simulink model "baseline_A_inference_v5"  (R2026a)
settings: Solver=FixedStepDiscrete  StartTime=0  StopTime=23  FixedStep=1
model workspace (MAT data in the model file):
  baseline_arch = 1
  baseline_inputs = timeseries
  baseline_inputs.Name = 'unnamed'
  baseline_inputs.DataInfo = tsdata.datametadata
  baseline_inputs.DataInfo.Interpolation = tsdata.interpolation
  baseline_inputs.DataInfo.Interpolation.Fhandle : function handle (value not decoded)
  baseline_inputs.DataInfo.Interpolation.Name = 'linear'
  baseline_inputs.TimeInfo = tsdata.timemetadata
  baseline_inputs.TimeInfo.Length = 24
  baseline_inputs.TimeInfo.DuplicateTimes = 0
  baseline_inputs.TimeInfo.Time_ = [0; 1; 2; 3; 4; 5; 6; 7; 8; 9; 10; 11; 12; 13; 14; 15; 16; 17; 18; 19; 20; 21; 22; 23]
  baseline_inputs.TimeInfo.Initialized = 1
  baseline_inputs.QualityInfo = tsdata.qualmetadata
  baseline_inputs.Data_ = [3026.659  81.2  1  2; 2218.177  78.3  1  2; 2902.304  81  1  2; 2193.91933333  77.9  1  2; 2808.14466667  81.3  1  2; 2120.17766667  75.1  1  2; 3824.575  80  1  2; 2700.98066667  75.7  1  2; 3026.659  81.2  1  3; 2205.66033333  74.9  1  3; 2902.304  81  1  3; 2112.29733333  72.9  1  3; 2808.14466667  81.3  1  3; 2092.628  71.7  1  3; 3824.575  80  1  3; 2542.90933333  73.8  1  3; 3026.659  81.2  1  4; 3382.50466667  75  1  4; 2902.304  81  1  4; 2413.05233333  73.3  1  4; 2808.14466667  81.3  1  4; 2538.15333333  73  1  4; 3824.575  80  1  4; 3938.38166667  73.7  1  4]
  baseline_mu = [2625.56568519 77.2222222222]
  baseline_p = [0.666654751449; 0.226875085596; -1.47953239563; 0.274529911025; -0.813940147404; -0.384768139912; 1.63750357072; -1.04590625677; 0.818587516624; -0.172278212697; -0.255378936098; -0.34034588768; 0; 0; 0; 0; 0; 0; 0; 0; 0; 0; 0; 0; 0; 0; 0; 0; 0; 0; 0; 0]
  baseline_sd = [585.088406321 4.03273116323]
Description:
  | Frozen A inference: linear/no-replay/seed101/stage3 demonstration with24 reporting views. Tick=record order, not physical time. Full30-checkpoint parity is in the separate result. No online learning.
settings Model: Creator=salih  LastModifiedBy=salih

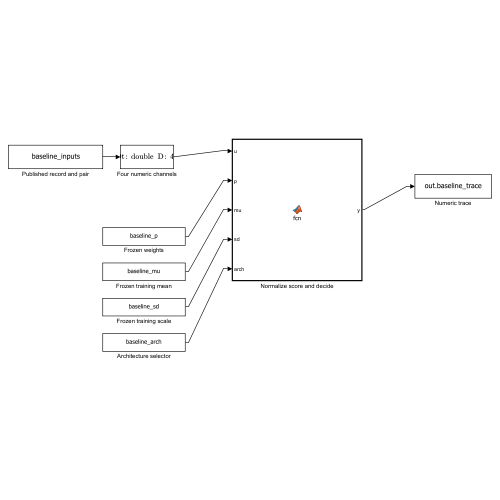
[thumbnail: Simulink's stored preview of the top-level diagram]
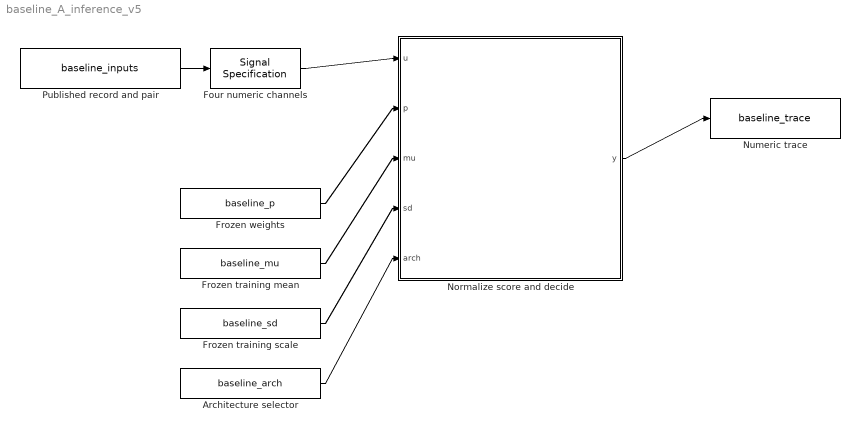
== system baseline_A_inference_v5 ==
  Architecture selector : Constant  Value=baseline_arch
  Four numeric channels : SignalSpecification  OutDataTypeStr=double  Dimensions=4
  Frozen training mean : Constant  Value=baseline_mu
  Frozen training scale : Constant  Value=baseline_sd
  Frozen weights : Constant  Value=baseline_p
  Normalize score and decide : MATLAB Function  TreatAsAtomicUnit=on
  Numeric trace : ToWorkspace  VariableName=baseline_trace  SampleTime=1
  Published record and pair : FromWorkspace  VariableName=baseline_inputs  SampleTime=1  Interpolate=off  OutputAfterFinalValue=Holding final value
  wires:
  Published record and pair/1 -> Four numeric channels/1
  Four numeric channels/1 -> Normalize score and decide/1(u)
  Frozen weights/1 -> Normalize score and decide/2(p)
  Frozen training mean/1 -> Normalize score and decide/3(mu)
  Frozen training scale/1 -> Normalize score and decide/4(sd)
  Architecture selector/1 -> Normalize score and decide/5(arch)
  Normalize score and decide/1(y) -> Numeric trace/1

== matlab function baseline_A_inference_v5/Normalize score and decide ==
  data: u input; y output; p input; mu input; sd input; arch input
function y = fcn(u,p,mu,sd,arch)
%#codegen
% u: [E_MPa, ShoreD, candidate_a, candidate_b]. Pair is control, not a feature.
% p: fixed32 parameter slots. arch1 linear; arch2 two-four-four tanh.
% y: Xnorm2, logits4, probabilities4, margin, forced, selected, status.
% status1 selected,0 nonselection,-1 failure. True label never enters here.
y=nan(1,14); y(12:13)=0; y(14)=-1;
if any(~isfinite(u(:))) || any(~isfinite(p(:))) || ...
        any(~isfinite(mu(:))) || any(~isfinite(sd(:))) || any(sd(:)<=0)
    return;
end
a=u(3); b=u(4);
if a~=1 || b~=floor(b) || b<2 || b>4 || (arch~=1 && arch~=2)
    return;
end
x=[(u(1)-mu(1))/sd(1),(u(2)-mu(2))/sd(2)];
if arch==1
    W=reshape(p(1:8),2,4); bias=reshape(p(9:12),1,4);
    z=x*W+bias;
else
    W1=reshape(p(1:8),2,4); b1=reshape(p(9:12),1,4);
    W2=reshape(p(13:28),4,4); b2=reshape(p(29:32),1,4);
    z=tanh(x*W1+b1)*W2+b2;
end
if any(~isfinite(z)), return; end
m=max(z(a),z(b)); ea=exp(z(a)-m); eb=exp(z(b)-m);
P=zeros(1,4); P(a)=ea/(ea+eb); P(b)=eb/(ea+eb);
margin=abs(P(a)-P(b)); forced=a;
if P(b)>P(a), forced=b; end % accepted pairs ascending; tie -> smallest index
selected=0; status=0;
if margin>=0.15 && P(a)~=P(b), selected=forced; status=1; end
y=[x,z,P,margin,forced,selected,status];
end
